simulink model "Motor_Models_Graduate_Version"  (R2024a)
settings: Solver=ode4  StartTime=0.0  StopTime=3  FixedStep=1/100  RelTol=1e-3  EnableMultiTasking=on
values from neighbouring files (symbols this model uses):
  Qvec = [-0.0101196491827 1.20927201569e-05 9.11792925381e-05 1.17252742353e-08 5.75013593968e-07 -0.000975617971472 2.07457043216e-13 -4.13179301718e-11 1.27812382623e-08 -8.38050058102e-06]    [PropData_16x55MR.mat]
undefined symbols (not defined in the file or in its folder): results_table, Vehicle
libraries: simulink_extras x1, slpidlib x1, aerolibanimutils x1
settings Model: xpc_rtwmakecfg_data=_xpciplib__xpcetherlib__xpcether8255xlib__xpcetherGbElib_  Creator=Omkar  LastModifiedBy=Teama
settings SolverCC: AlgebraicLoopSolver=TrustRegion  AutoInsertRateTranBlk=on
settings DataIOCC: ReturnWorkspaceOutputs=off
settings DebuggingCC: UnderSpecifiedDataTypeMsg=warning  UnconnectedInputMsg=warning  UnconnectedOutputMsg=warning  UnconnectedLineMsg=warning  UnderSpecifiedDimensionMsg=warning  ArithmeticOperatorsInVariantConditions=warning
settings ModelReferenceCC: EnableRefExpFcnMdlSchedulingChecks=on
settings SFSimCC: SimUseLocalCustomCode=off  CustomCodeUndefinedFunction=UseInterfaceOnly
settings RTWCC: RTWUseLocalCustomCode=off  GPUComputeCapability=3.5  DLArmComputeVersion=19.05

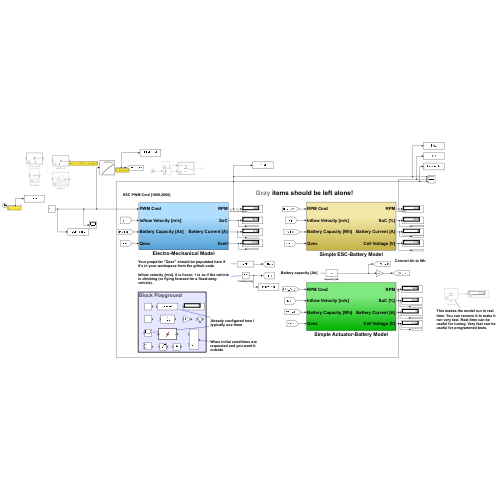
[thumbnail: Simulink's stored preview of the top-level diagram]
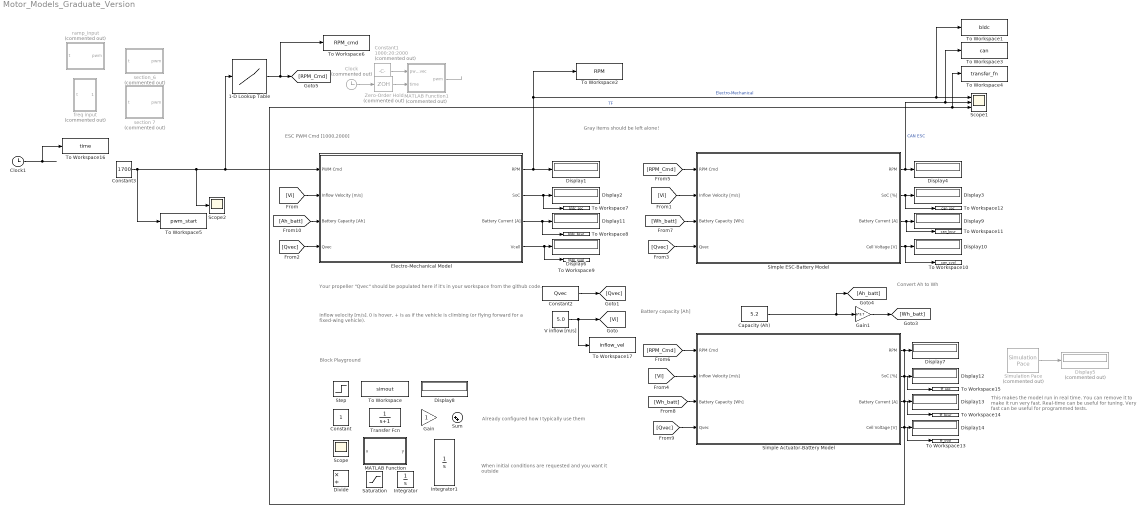
== system Motor_Models_Graduate_Version ==
  note: Block Playground
  note: Inflow velocity [m/s]. 0 is hover, + is as if the vehicle is climbing (or flying forward for a fixed-wing vehicle).
  note: Gray items should be left alone!
  note: Your propeller "Qvec" should be populated here if it's in your workspace from the github code.
  note: Battery capacity [Ah]
  note: ESC PWM Cmd [1000,2000]
  note: Already configured how I typically use them
  note: When initial conditions are requested and you want it outside
  note: This makes the model run in real time. You can remove it to make it run very fast. Real-time can be useful for tuning. Very fast can be useful for programmed tests.
  note: Convert Ah to Wh
  1-D Lookup Table : Lookup_n-D  NumberOfTableDimensions=1  BreakpointsForDimension1=results_table.pwm  Table=results_table.RPM  InternalRulePriority=Speed  RndMeth=Simplest
  Capacity (Ah) : Constant  Value=5.2
  Clock : Clock  Commented=on
  Clock1 : Clock
  Constant : Constant
  Constant1 : Constant  Commented=on  Value=1000:20:2000
  Constant2 : Constant  Value=Qvec
  Constant3 : Constant  Value=1700
  Display{1..4,6..14} (13 alike) : Display
  Display5 : Display  Commented=on
  Divide : Product  Inputs=*/
  Electro-Mechanical Model : Subsystem
  Gain : Gain
  Gain1 : Gain  Gain=6*3.7
  Integrator : Integrator
  Integrator1 : Integrator  InitialConditionSource=external
  MATLAB Function : MATLAB Function  TreatAsAtomicUnit=on
  MATLAB Function1 : MATLAB Function  Commented=on  TreatAsAtomicUnit=on
  Saturation : Saturate
  Scope : Scope
  Scope1 : Scope  NumInputPorts=3
  Scope2 : Scope
  Simple Actuator-Battery Model : Subsystem
  Simple ESC-Battery Model : Subsystem
  Simulation Pace : aerolibanimutils/Simulation Pace  Commented=on  SimulationPace=1  SleepMode=Auto  OutputPaceError=on  SampleTime=-1
  Step : Step  SampleTime=0
  Sum : Sum  Inputs=|++
  To Workspace : ToWorkspace  VariableName=simout  SampleTime=-1
      settings: Save2DSignal=2-D array (concatenate along first dimension)
  To Workspace1 : ToWorkspace  VariableName=bldc  SampleTime=-1
      settings: Save2DSignal=2-D array (concatenate along first dimension)
  To Workspace10 : ToWorkspace  VariableName=can_cvol  SampleTime=-1
      settings: Save2DSignal=2-D array (concatenate along first dimension)
  To Workspace11 : ToWorkspace  VariableName=can_bcur  SampleTime=-1
      settings: Save2DSignal=2-D array (concatenate along first dimension)
  To Workspace12 : ToWorkspace  VariableName=can_soc  SampleTime=-1
      settings: Save2DSignal=2-D array (concatenate along first dimension)
  To Workspace13 : ToWorkspace  VariableName=tf_cvol  SampleTime=-1
      settings: Save2DSignal=2-D array (concatenate along first dimension)
  To Workspace14 : ToWorkspace  VariableName=tf_bcur  SampleTime=-1
      settings: Save2DSignal=2-D array (concatenate along first dimension)
  To Workspace15 : ToWorkspace  VariableName=tf_soc  SampleTime=-1
      settings: Save2DSignal=2-D array (concatenate along first dimension)
  To Workspace16 : ToWorkspace  VariableName=time  SampleTime=-1
      settings: Save2DSignal=2-D array (concatenate along first dimension)
  To Workspace17 : ToWorkspace  VariableName=inflow_vel  SampleTime=-1
      settings: Save2DSignal=2-D array (concatenate along first dimension)
  To Workspace2 : ToWorkspace  VariableName=RPM  SampleTime=-1
      settings: Save2DSignal=2-D array (concatenate along first dimension)
  To Workspace3 : ToWorkspace  VariableName=can  SampleTime=-1
      settings: Save2DSignal=2-D array (concatenate along first dimension)
  To Workspace4 : ToWorkspace  VariableName=transfer_fn  SampleTime=-1
      settings: Save2DSignal=2-D array (concatenate along first dimension)
  To Workspace5 : ToWorkspace  VariableName=pwm_start  SampleTime=-1
      settings: Save2DSignal=2-D array (concatenate along first dimension)
  To Workspace6 : ToWorkspace  VariableName=RPM_cmd
      settings: Save2DSignal=2-D array (concatenate along first dimension)
  To Workspace7 : ToWorkspace  VariableName=bldc_soc  SampleTime=-1
      settings: Save2DSignal=2-D array (concatenate along first dimension)
  To Workspace8 : ToWorkspace  VariableName=bldc_bcur  SampleTime=-1
      settings: Save2DSignal=2-D array (concatenate along first dimension)
  To Workspace9 : ToWorkspace  VariableName=bldc_cvol  SampleTime=-1
      settings: Save2DSignal=2-D array (concatenate along first dimension)
  Transfer Fcn : TransferFcn  Denominator=[1 1]
  V inflow [m/s] : Constant  Value=5.0
  Zero-Order Hold : ZeroOrderHold  Commented=on  SampleTime=-1
  freq input : Subsystem  Commented=on
  ramp_input : MATLAB Function  Commented=on  TreatAsAtomicUnit=on
  section 7 : Subsystem  Commented=on
  section_6 : MATLAB Function  Commented=on  TreatAsAtomicUnit=on
  wires:
  Simulation Pace/1 -> Display5/1
  Electro-Mechanical Model/1(RPM) -> To Workspace1/1, Scope1/1, To Workspace2/1, Display1/1  "Electro-Mechanical"
  Electro-Mechanical Model/2(SoC) -> To Workspace7/1, Display2/1
  [RPM_Cmd] -> Simple ESC-Battery Model/1(RPM Cmd)
  Simple ESC-Battery Model/1(RPM) -> To Workspace3/1, Scope1/2, Display4/1  "CAN ESC"
  Simple ESC-Battery Model/2(SoC [%]) -> To Workspace12/1, Display3/1
  Electro-Mechanical Model/4(Vcell) -> To Workspace9/1, Display6/1
  V inflow [m/s]/1 -> To Workspace17/1, [Vi]
  [Vi] -> Electro-Mechanical Model/2(Inflow Velocity [m/s])
  [Vi] -> Simple ESC-Battery Model/2(Inflow Velocity [m/s])
  Constant2/1 -> [Qvec]
  [Qvec] -> Electro-Mechanical Model/4(Qvec)
  [Qvec] -> Simple ESC-Battery Model/4(Qvec)
  Simple ESC-Battery Model/3(Battery Current [A]) -> To Workspace11/1, Display9/1
  Simple ESC-Battery Model/4(Cell Voltage [V]) -> To Workspace10/1, Display10/1
  [RPM_Cmd] -> Simple Actuator-Battery Model/1(RPM Cmd)
  [Vi] -> Simple Actuator-Battery Model/2(Inflow Velocity [m/s])
  Capacity (Ah)/1 -> Gain1/1, [Ah_batt]
  [Wh_batt] -> Simple ESC-Battery Model/3(Battery Capacity [Wh])
  [Wh_batt] -> Simple Actuator-Battery Model/3(Battery Capacity [Wh])
  [Qvec] -> Simple Actuator-Battery Model/4(Qvec)
  Gain1/1 -> [Wh_batt]
  [Ah_batt] -> Electro-Mechanical Model/3(Battery Capacity [Ah])
  Simple Actuator-Battery Model/1(RPM) -> To Workspace4/1, Scope1/3, Display7/1  "TF"
  Electro-Mechanical Model/3(Battery Current [A]) -> To Workspace8/1, Display11/1
  Simple Actuator-Battery Model/2(SoC [%]) -> To Workspace15/1, Display12/1
  Simple Actuator-Battery Model/3(Battery Current [A]) -> To Workspace14/1, Display13/1
  Simple Actuator-Battery Model/4(Cell Voltage [V]) -> To Workspace13/1, Display14/1
  Constant1/1 -> MATLAB Function1/1(pwm_vec)
  MATLAB Function1/1(pwm) -> ?
  Clock/1 -> Zero-Order Hold/1
  Zero-Order Hold/1 -> MATLAB Function1/2(time)
  Clock1/1 -> To Workspace16/1
  Constant3/1 -> To Workspace5/1, Scope2/1, 1-D Lookup Table/1, Electro-Mechanical Model/1(PWM Cmd)
  1-D Lookup Table/1 -> To Workspace6/1, [RPM_Cmd]

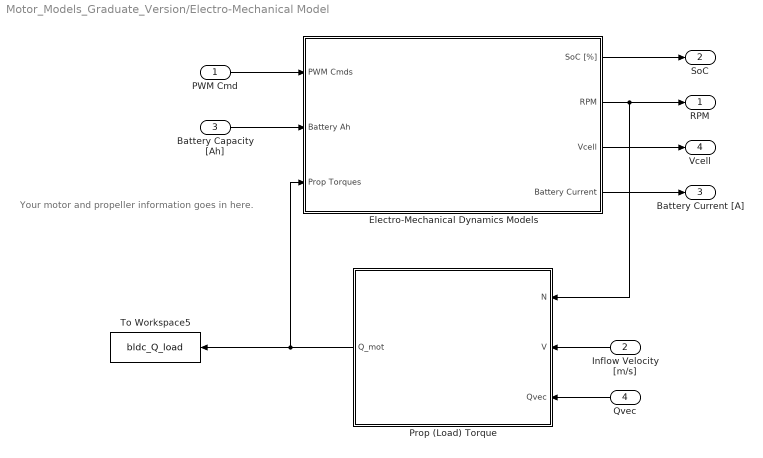
== system Motor_Models_Graduate_Version/Electro-Mechanical Model ==
  note: Your motor and propeller information goes in here.
  PWM Cmd : Inport
  Inflow Velocity [m/s] : Inport  Port=2
  Battery Capacity [Ah] : Inport  Port=3
  Qvec : Inport  Port=4
  Electro-Mechanical Dynamics Models : Subsystem
  Prop (Load) Torque : MATLAB Function  TreatAsAtomicUnit=on
  To Workspace5 : ToWorkspace  VariableName=bldc_Q_load  SampleTime=-1
      settings: Save2DSignal=2-D array (concatenate along first dimension)
  RPM : Outport
  SoC : Outport  Port=2
  Battery Current [A] : Outport  Port=3
  Vcell : Outport  Port=4
  wires:
  Prop (Load) Torque/1(Q_mot) -> To Workspace5/1, Electro-Mechanical Dynamics Models/3(Prop Torques)
  Qvec/1 -> Prop (Load) Torque/3(Qvec)
  Electro-Mechanical Dynamics Models/2(RPM) -> Prop (Load) Torque/1(N), RPM/1
  Electro-Mechanical Dynamics Models/1(SoC [%]) -> SoC/1
  PWM Cmd/1 -> Electro-Mechanical Dynamics Models/1(PWM Cmds)
  Inflow Velocity [m/s]/1 -> Prop (Load) Torque/2(V)
  Electro-Mechanical Dynamics Models/3(Vcell) -> Vcell/1
  Battery Capacity [Ah]/1 -> Electro-Mechanical Dynamics Models/2(Battery Ah)
  Electro-Mechanical Dynamics Models/4(Battery Current) -> Battery Current [A]/1

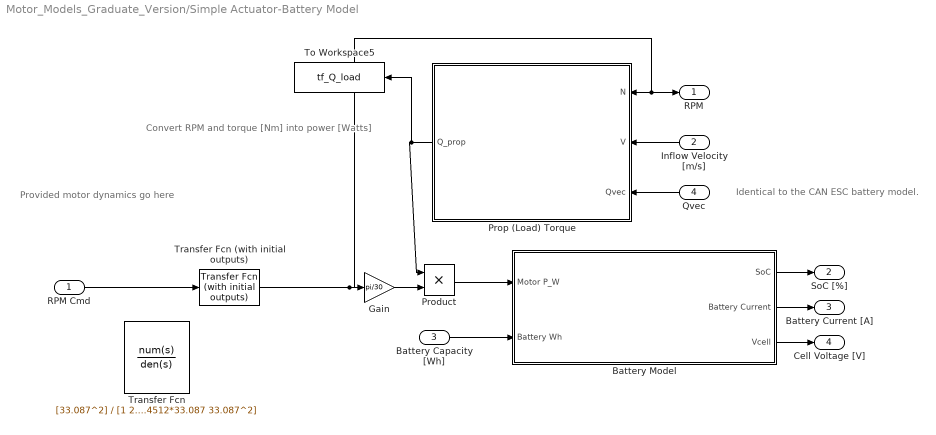
== system Motor_Models_Graduate_Version/Simple Actuator-Battery Model ==
  note: Identical to the CAN ESC battery model.
  note: Provided motor dynamics go here
  note: Convert RPM and torque [Nm] into power [Watts]
  RPM Cmd : Inport
  Inflow Velocity [m/s] : Inport  Port=2
  Battery Capacity [Wh] : Inport  Port=3
  Qvec : Inport  Port=4
  Battery Model : Subsystem
  Gain : Gain  Gain=pi/30
  Product : Product
  Prop (Load) Torque : MATLAB Function  TreatAsAtomicUnit=on
  To Workspace5 : ToWorkspace  VariableName=tf_Q_load  SampleTime=-1
      settings: Save2DSignal=2-D array (concatenate along first dimension)
  Transfer Fcn : TransferFcn  Numerator=[33.087^2]  Denominator=[1 2*1.4512*33.087 33.087^2]
  Transfer Fcn (with initial outputs) : simulink_extras/Additional Linear/Transfer Fcn (with initial outputs)  N=[33.087^2]  D=[1 2*1.4512*33.087 33.087^2]  Y0=0  U0=0
  RPM : Outport
  SoC [%] : Outport  Port=2
  Battery Current [A] : Outport  Port=3
  Cell Voltage [V] : Outport  Port=4
  wires:
  Battery Model/3(Vcell) -> Cell Voltage [V]/1
  Prop (Load) Torque/1(Q_prop) -> To Workspace5/1, Product/1
  Battery Model/2(Battery Current) -> Battery Current [A]/1
  Qvec/1 -> Prop (Load) Torque/3(Qvec)
  Inflow Velocity [m/s]/1 -> Prop (Load) Torque/2(V)
  Battery Model/1(SoC) -> SoC [%]/1
  Transfer Fcn (with initial outputs)/1 -> RPM/1, Prop (Load) Torque/1(N), Gain/1
  Product/1 -> Battery Model/1(Motor P_W)
  Battery Capacity [Wh]/1 -> Battery Model/2(Battery Wh)
  RPM Cmd/1 -> Transfer Fcn (with initial outputs)/1
  Gain/1 -> Product/2

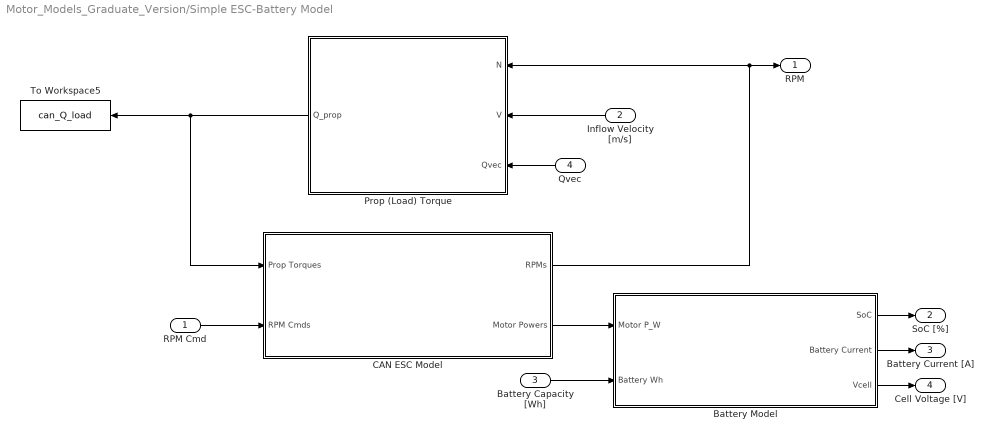
== system Motor_Models_Graduate_Version/Simple ESC-Battery Model ==
  RPM Cmd : Inport
  Inflow Velocity [m/s] : Inport  Port=2
  Battery Capacity [Wh] : Inport  Port=3
  Qvec : Inport  Port=4
  Battery Model : Subsystem
  CAN ESC Model : Subsystem
  Prop (Load) Torque : MATLAB Function  TreatAsAtomicUnit=on
  To Workspace5 : ToWorkspace  VariableName=can_Q_load  SampleTime=-1
      settings: Save2DSignal=2-D array (concatenate along first dimension)
  RPM : Outport
  SoC [%] : Outport  Port=2
  Battery Current [A] : Outport  Port=3
  Cell Voltage [V] : Outport  Port=4
  wires:
  Battery Capacity [Wh]/1 -> Battery Model/2(Battery Wh)
  CAN ESC Model/2(Motor Powers) -> Battery Model/1(Motor P_W)
  CAN ESC Model/1(RPMs) -> RPM/1, Prop (Load) Torque/1(N)
  Battery Model/1(SoC) -> SoC [%]/1
  Inflow Velocity [m/s]/1 -> Prop (Load) Torque/2(V)
  Qvec/1 -> Prop (Load) Torque/3(Qvec)
  Battery Model/2(Battery Current) -> Battery Current [A]/1
  Prop (Load) Torque/1(Q_prop) -> To Workspace5/1, CAN ESC Model/1(Prop Torques)
  RPM Cmd/1 -> CAN ESC Model/2(RPM Cmds)
  Battery Model/3(Vcell) -> Cell Voltage [V]/1

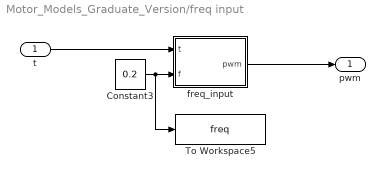
== system Motor_Models_Graduate_Version/freq input ==
  t : Inport
  Constant3 : Constant  Value=0.2
  To Workspace5 : ToWorkspace  VariableName=freq  SampleTime=-1
      settings: Save2DSignal=2-D array (concatenate along first dimension)
  freq_input : MATLAB Function  TreatAsAtomicUnit=on
  pwm : Outport
  wires:
  Constant3/1 -> To Workspace5/1, freq_input/2(f)
  freq_input/1(pwm) -> pwm/1
  t/1 -> freq_input/1(t)

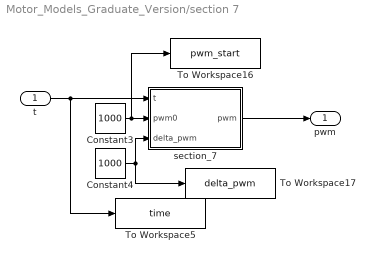
== system Motor_Models_Graduate_Version/section 7 ==
  t : Inport
  Constant3 : Constant  Value=1000
  Constant4 : Constant  Value=1000
  To Workspace16 : ToWorkspace  VariableName=pwm_start  SampleTime=-1
      settings: Save2DSignal=2-D array (concatenate along first dimension)
  To Workspace17 : ToWorkspace  VariableName=delta_pwm  SampleTime=-1
      settings: Save2DSignal=2-D array (concatenate along first dimension)
  To Workspace5 : ToWorkspace  VariableName=time  SampleTime=-1
      settings: Save2DSignal=2-D array (concatenate along first dimension)
  section_7 : MATLAB Function  TreatAsAtomicUnit=on
  pwm : Outport
  wires:
  t/1 -> section_7/1(t), To Workspace5/1
  section_7/1(pwm) -> pwm/1
  Constant4/1 -> section_7/3(delta_pwm), To Workspace17/1
  Constant3/1 -> To Workspace16/1, section_7/2(pwm0)

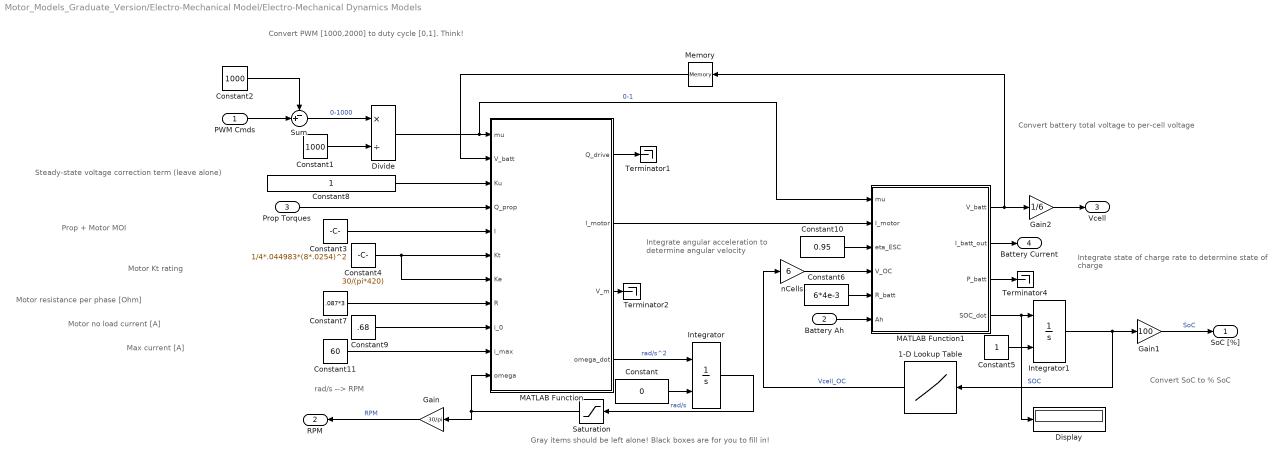
== system Motor_Models_Graduate_Version/Electro-Mechanical Model/Electro-Mechanical Dynamics Models ==
  note: Gray items should be left alone!
      | Black boxes are for you to fill in!
  note: Convert battery total voltage to per-cell voltage
  note: Integrate state of charge rate to determine state of charge
  note: Steady-state voltage correction term (leave alone)
  note: Convert PWM [1000,2000] to duty cycle [0,1]. Think!
  note: Prop + Motor MOI
  note: Motor Kt rating
  note: Motor resistance per phase [Ohm]
  note: Motor no load current [A]
  note: Max current [A]
  note: Integrate angular acceleration to determine angular velocity
  note: Convert SoC to % SoC
  note: rad/s --> RPM
  PWM Cmds : Inport
  Battery Ah : Inport  Port=2
  Prop Torques : Inport  Port=3
  1-D Lookup Table : Lookup_n-D  NumberOfTableDimensions=1  BreakpointsForDimension1="[0    0.05  0.10  0.20  0.30  0.40  0.50  0.60  0.70  0.80  0.90  1.00]"  Table="[3.20 3.45  3.55  3.65  3.70  3.74  3.77  3.80  3.84  3.90  4.00  4.20]"  InternalRulePriority=Speed  RndMeth=Simplest
  Constant : Constant  Value=0
  Constant1 : Constant  Value=1000
  Constant10 : Constant  Value=0.95
  Constant11 : Constant  Value=60
  Constant2 : Constant  Value=1000
  Constant3 : Constant  Value=1/4*.044983*(8*.0254)^2
  Constant4 : Constant  Value=30/(pi*420)
  Constant5 : Constant
  Constant6 : Constant  Value=6*4e-3
  Constant7 : Constant  Value=.087*3
  Constant8 : Constant
  Constant9 : Constant  Value=.68
  Display : Display
  Divide : Product  Inputs=*/
  Gain : Gain  Gain=30/pi
  Gain1 : Gain  Gain=100
  Gain2 : Gain  Gain=1/6
  Integrator : Integrator  InitialConditionSource=external
  Integrator1 : Integrator  InitialConditionSource=external
  MATLAB Function : MATLAB Function  TreatAsAtomicUnit=on
  MATLAB Function1 : MATLAB Function  TreatAsAtomicUnit=on
  Memory : Memory  InitialCondition=25.2
  Saturation : Saturate  UpperLimit=inf  LowerLimit=0
  Sum : Sum  Inputs=-+|
  Terminator1 : Terminator
  Terminator2 : Terminator
  Terminator4 : Terminator
  nCells : Gain  Gain=6
  SoC [%] : Outport
  RPM : Outport  Port=2
  Vcell : Outport  Port=3
  Battery Current : Outport  Port=4
  wires:
  Battery Ah/1 -> MATLAB Function1/6(Ah)
  MATLAB Function1/4(SOC_dot) -> Display/1, Integrator1/1
  Divide/1 -> MATLAB Function1/1(mu), MATLAB Function/1(mu)  "0-1"
  Integrator/1 -> Saturation/1  "rad/s"
  Constant10/1 -> MATLAB Function1/3(eta_ESC)
  Integrator1/1 -> Gain1/1, 1-D Lookup Table/1  "SOC"
  Constant3/1 -> MATLAB Function/5(I)
  Constant/1 -> Integrator/2
  Constant6/1 -> MATLAB Function1/5(R_batt)
  MATLAB Function/4(omega_dot) -> Integrator/1  "rad/s^2"
  nCells/1 -> MATLAB Function1/4(V_OC)
  MATLAB Function/3(V_m) -> Terminator2/1
  1-D Lookup Table/1 -> nCells/1  "Vcell_OC"
  Constant5/1 -> Integrator1/2
  Prop Torques/1 -> MATLAB Function/4(Q_prop)
  Constant4/1 -> MATLAB Function/7(Ke), MATLAB Function/6(Kt)
  Constant7/1 -> MATLAB Function/8(R)
  Constant9/1 -> MATLAB Function/9(i_0)
  Constant11/1 -> MATLAB Function/10(i_max)
  Gain/1 -> RPM/1  "RPM"
  Constant8/1 -> MATLAB Function/3(Ku)
  Sum/1 -> Divide/1  "0-1000"
  Constant1/1 -> Divide/2
  Constant2/1 -> Sum/1
  PWM Cmds/1 -> Sum/2
  Gain1/1 -> SoC [%]/1  "SoC"
  MATLAB Function/2(I_motor) -> MATLAB Function1/2(I_motor)
  MATLAB Function1/3(P_batt) -> Terminator4/1
  MATLAB Function1/1(V_batt) -> Gain2/1, Memory/1
  MATLAB Function/1(Q_drive) -> Terminator1/1
  Gain2/1 -> Vcell/1
  MATLAB Function1/2(I_batt_out) -> Battery Current/1
  Memory/1 -> MATLAB Function/2(V_batt)
  Saturation/1 -> Gain/1, MATLAB Function/11(omega)

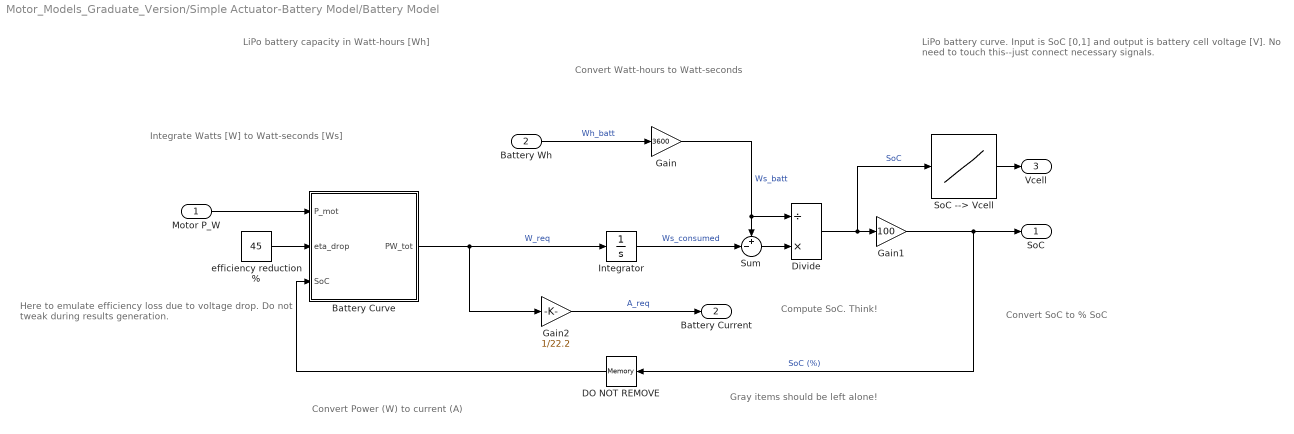
== system Motor_Models_Graduate_Version/Simple Actuator-Battery Model/Battery Model ==
  note: Gray items should be left alone!
  note: Integrate Watts [W] to Watt-seconds [Ws]
  note: Here to emulate efficiency loss due to voltage drop. Do not tweak during results generation.
  note: Convert Power (W) to current (A)
  note: Convert SoC to % SoC
  note: Convert Watt-hours to Watt-seconds
  note: LiPo battery capacity in Watt-hours [Wh]
  note: LiPo battery curve. Input is SoC [0,1] and output is battery cell voltage [V]. No need to touch this--just connect necessary signals.
  note: Compute SoC. Think!
  Motor P_W : Inport
  Battery Wh : Inport  Port=2
  Battery Curve : MATLAB Function  TreatAsAtomicUnit=on
  DO NOT REMOVE : Memory  InitialCondition=100
  Divide : Product  Inputs=/*
  Gain : Gain  Gain=3600
  Gain1 : Gain  Gain=100
  Gain2 : Gain  Gain=1/22.2
  Integrator : Integrator
  SoC --> Vcell : Lookup_n-D  NumberOfTableDimensions=1  BreakpointsForDimension1="[0    0.05  0.10  0.20  0.30  0.40  0.50  0.60  0.70  0.80  0.90  1.00]"  Table="[3.20 3.45  3.55  3.65  3.70  3.74  3.77  3.80  3.84  3.90  4.00  4.20]"  InternalRulePriority=Speed  RndMeth=Simplest
  Sum : Sum  Inputs=+-|
  efficiency reduction % : Constant  Value=45
  SoC : Outport
  Battery Current : Outport  Port=2
  Vcell : Outport  Port=3
  wires:
  SoC --> Vcell/1 -> Vcell/1
  Gain2/1 -> Battery Current/1  "A_req"
  efficiency reduction %/1 -> Battery Curve/2(eta_drop)
  DO NOT REMOVE/1 -> Battery Curve/3(SoC)
  Battery Curve/1(PW_tot) -> Gain2/1, Integrator/1  "W_req"
  Gain/1 -> Divide/1, Sum/1  "Ws_batt"
  Gain1/1 -> SoC/1, DO NOT REMOVE/1  "SoC (%)"
  Divide/1 -> SoC --> Vcell/1, Gain1/1  "SoC"
  Integrator/1 -> Sum/2  "Ws_consumed"
  Sum/1 -> Divide/2
  Motor P_W/1 -> Battery Curve/1(P_mot)
  Battery Wh/1 -> Gain/1  "Wh_batt"

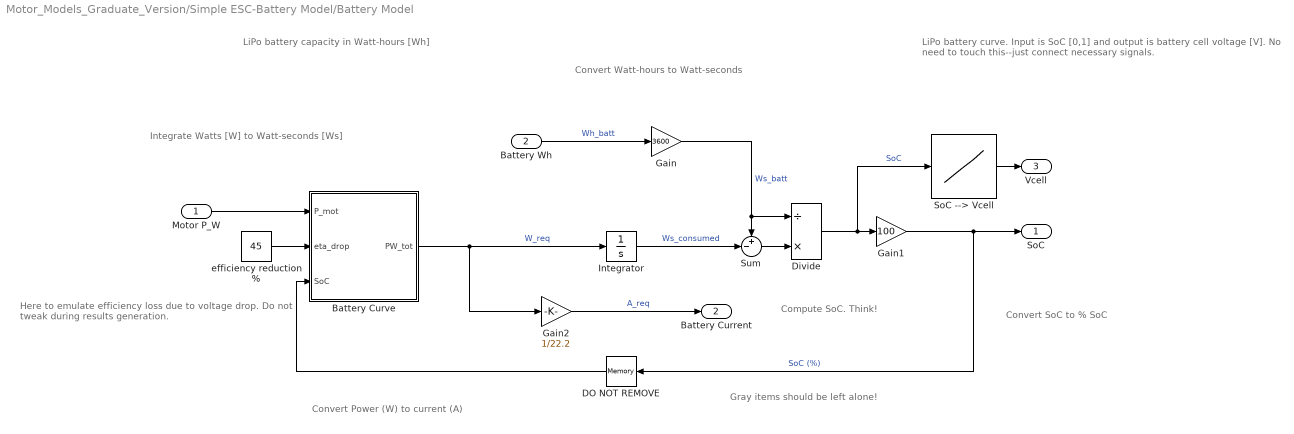
== system Motor_Models_Graduate_Version/Simple ESC-Battery Model/Battery Model ==
  note: Gray items should be left alone!
  note: Integrate Watts [W] to Watt-seconds [Ws]
  note: Here to emulate efficiency loss due to voltage drop. Do not tweak during results generation.
  note: Convert Power (W) to current (A)
  note: Convert SoC to % SoC
  note: Convert Watt-hours to Watt-seconds
  note: LiPo battery capacity in Watt-hours [Wh]
  note: LiPo battery curve. Input is SoC [0,1] and output is battery cell voltage [V]. No need to touch this--just connect necessary signals.
  note: Compute SoC. Think!
  Motor P_W : Inport
  Battery Wh : Inport  Port=2
  Battery Curve : MATLAB Function  TreatAsAtomicUnit=on
  DO NOT REMOVE : Memory  InitialCondition=100
  Divide : Product  Inputs=/*
  Gain : Gain  Gain=3600
  Gain1 : Gain  Gain=100
  Gain2 : Gain  Gain=1/22.2
  Integrator : Integrator
  SoC --> Vcell : Lookup_n-D  NumberOfTableDimensions=1  BreakpointsForDimension1="[0    0.05  0.10  0.20  0.30  0.40  0.50  0.60  0.70  0.80  0.90  1.00]"  Table="[3.20 3.45  3.55  3.65  3.70  3.74  3.77  3.80  3.84  3.90  4.00  4.20]"  InternalRulePriority=Speed  RndMeth=Simplest
  Sum : Sum  Inputs=+-|
  efficiency reduction % : Constant  Value=45
  SoC : Outport
  Battery Current : Outport  Port=2
  Vcell : Outport  Port=3
  wires:
  SoC --> Vcell/1 -> Vcell/1
  Gain2/1 -> Battery Current/1  "A_req"
  efficiency reduction %/1 -> Battery Curve/2(eta_drop)
  DO NOT REMOVE/1 -> Battery Curve/3(SoC)
  Battery Curve/1(PW_tot) -> Gain2/1, Integrator/1  "W_req"
  Gain/1 -> Divide/1, Sum/1  "Ws_batt"
  Gain1/1 -> SoC/1, DO NOT REMOVE/1  "SoC (%)"
  Divide/1 -> SoC --> Vcell/1, Gain1/1  "SoC"
  Integrator/1 -> Sum/2  "Ws_consumed"
  Sum/1 -> Divide/2
  Motor P_W/1 -> Battery Curve/1(P_mot)
  Battery Wh/1 -> Gain/1  "Wh_batt"

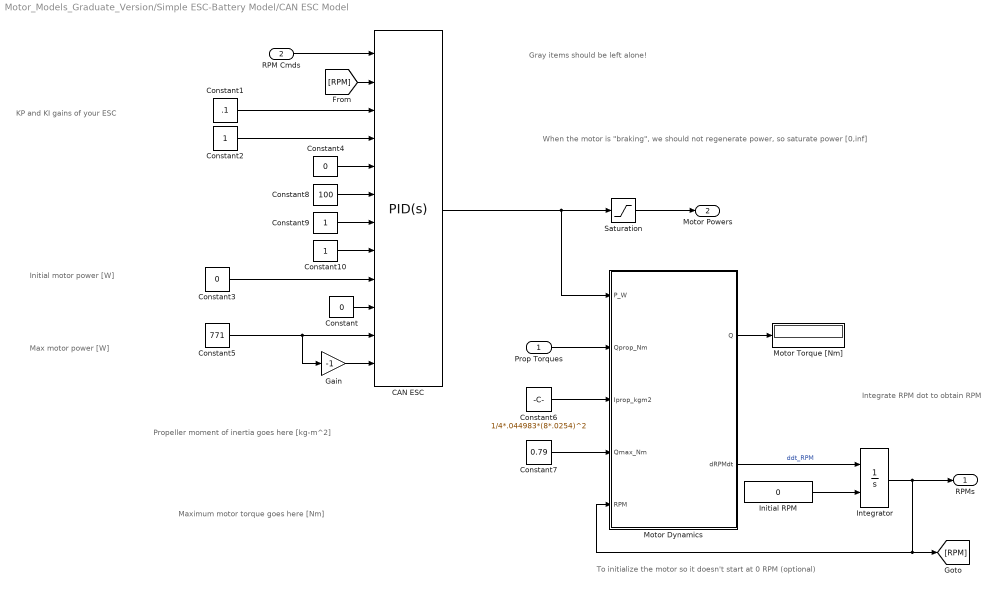
== system Motor_Models_Graduate_Version/Simple ESC-Battery Model/CAN ESC Model ==
  note: Propeller moment of inertia goes here [kg-m^2]
  note: Maximum motor torque goes here [Nm]
  note: To initialize the motor so it doesn't start at 0 RPM (optional)
  note: Max motor power [W]
  note: Initial motor power [W]
  note: KP and KI gains
      | of your ESC
  note: Gray items should be left alone!
  note: When the motor is "braking", we should not regenerate power, so saturate power [0,inf]
  note: Integrate RPM dot to obtain RPM
  Prop Torques : Inport
  RPM Cmds : Inport  Port=2
  CAN ESC : slpidlib/PID Controller (2DOF)  Controller=PID  Form=Parallel  TimeDomain=Continuous-time  UseExternalTs=off  SampleTime=-1  IntegratorMethod=Forward Euler  FilterMethod=Forward Euler  ControllerParametersSource=external  P=Vehicle.Controls.ESC.KP_LP  I=Vehicle.Controls.ESC.KI_LP  UseKiTs=off  D=0  UseExternalDerivativeSource=off  N=100  UseFilter=on  b=1  c=0  TunerSelectOption=Transfer Function Based (PID Tuner App)  InitialConditionSource=external  InitialConditionForIntegrator=0  InitialConditionForFilter=0  DifferentiatorICPrevScaledInput=0  ExternalReset=none  TrackingMode=off  Kt=1  LimitOutput=on  SatLimitsSource=external  UpperSaturationLimit=16e3  LowerSaturationLimit=-16e3  LinearizeAsGain=on  AntiWindupMode=clamping  Kb=1  LimitIntegrator=off  UpperIntegratorSaturationLimit=inf  LowerIntegratorSaturationLimit=-inf  POutMin=[]  POutMax=[]  IOutMin=[]  IOutMax=[]  DOutMin=[]  DOutMax=[]  NOutMin=[]  NOutMax=[]  bOutMin=[]  bOutMax=[]  cOutMin=[]  cOutMax=[]  SumOutMin=[]  SumOutMax=[]  SaturationOutMin=[]  SaturationOutMax=[]  PParamMin=[]  PParamMax=[]  IParamMin=[]  IParamMax=[]  DParamMin=[]  DParamMax=[]  NParamMin=[]  NParamMax=[]  bParamMin=[]  bParamMax=[]  cParamMin=[]  cParamMax=[]  KbParamMin=[]  KbParamMax=[]  KtParamMin=[]  KtParamMax=[]  KbOutMin=[]  KbOutMax=[]  KtOutMin=[]  KtOutMax=[]  IntegratorOutMin=[]  IntegratorOutMax=[]  FilterOutMin=[]  FilterOutMax=[]  SumI1OutMin=[]  SumI1OutMax=[]  SumI2OutMin=[]  SumI2OutMax=[]  SumI3OutMin=[]  SumI3OutMax=[]  SumI4OutMin=[]  SumI4OutMax=[]  SumDOutMin=[]  SumDOutMax=[]  Sum1OutMin=[]  Sum1OutMax=[]  Sum2OutMin=[]  Sum2OutMax=[]  Sum3OutMin=[]  Sum3OutMax=[]  DifferentiatorOutMin=[]  DifferentiatorOutMax=[]  FilterDiffOutCoefMin=[]  FilterDiffOutCoefMax=[]  ReciprocalOutMin=[]  ReciprocalOutMax=[]  SumDenOutMin=[]  SumDenOutMax=[]  SumNumOutMin=[]  SumNumOutMax=[]  DivideOutMin=[]  DivideOutMax=[]  UdiffTsProdOutMin=[]  UdiffTsProdOutMax=[]  NTsProdOutMin=[]  NTsProdOutMax=[]  UintegralTsProdOutMin=[]  UintegralTsProdOutMax=[]  UngainTsProdOutMin=[]  UngainTsProdOutMax=[]  ClampingZeroOutDataTypeStr=Inherit: Inherit via back propagation  ClampingZeroOutMin=[]  ClampingZeroOutMax=[]  FilterDenConstantOutDataTypeStr=Inherit: Inherit via back propagation  FilterDenConstantOutMin=[]  FilterDenConstantOutMax=[]  PCopyOutDataTypeStr=Inherit: Inherit via back propagation  PCopyOutMin=[]  PCopyOutMax=[]  NCopyOutDataTypeStr=Inherit: Inherit via back propagation  NCopyOutMin=[]  NCopyOutMax=[]  IntegratorContinuousStateAttributes=''  IntegratorStateMustResolveToSignalObject=off  IntegratorRTWStateStorageClass=Auto  FilterContinuousStateAttributes=''  FilterStateMustResolveToSignalObject=off  FilterRTWStateStorageClass=Auto  ParallelPVariant=ExternalParameters  IdealPVariant=Disabled  IVariant=ExternalParameters  DVariant=ExternalParameters  bVariant=ExternalParameters  cVariant=ExternalParameters  IntegratorVariant=Continuous  SatVariant=External  AWVariant=ContClampingParallel  PCopyVariant=Disabled  TRVariant=Disabled  FdbkBlocksVariant=Forward  IdealPFdbkVariant=Disabled  SatFdbkVariant=Disabled  DerivativeFilterVariant=ContFilter  NVariant=ExternalParameters  NCopyVariant=Disabled  FilterICVariant=ExternalICs  IntegratorICVariant=ExternalICs  ExternalResetVariant=Disabled  TRSumVariant=Passthrough  SumFdbkVariant=Disabled  SumVariant=Sum_PID  TsampFilterVariant=InternalTs  TsampNgainVariant=Passthrough  TsampIntegralVariant=Disabled_SignalSpec  ExternalSaturationOutDataTypeStr=Inherit: Same as second input  DerivativeSourceVariant=ErrorSignal
  Constant : Constant  Value=0
  Constant1 : Constant  Value=.1
  Constant10 : Constant
  Constant2 : Constant
  Constant3 : Constant  Value=0
  Constant4 : Constant  Value=0
  Constant5 : Constant  Value=771
  Constant6 : Constant  Value=1/4*.044983*(8*.0254)^2
  Constant7 : Constant  Value=0.79
  Constant8 : Constant  Value=100
  Constant9 : Constant
  Gain : Gain  Gain=-1
  Initial RPM : Constant  Value=0
  Integrator : Integrator  InitialConditionSource=external
  Motor Dynamics : MATLAB Function  TreatAsAtomicUnit=on
  Motor Torque [Nm] : Display
  Saturation : Saturate  UpperLimit=inf  LowerLimit=0
  RPMs : Outport
  Motor Powers : Outport  Port=2
  wires:
  Constant/1 -> CAN ESC/10
  Constant3/1 -> CAN ESC/9
  Integrator/1 -> Motor Dynamics/5(RPM), [RPM], RPMs/1
  RPM Cmds/1 -> CAN ESC/1
  Constant7/1 -> Motor Dynamics/4(Qmax_Nm)
  Prop Torques/1 -> Motor Dynamics/2(Qprop_Nm)
  Initial RPM/1 -> Integrator/2
  Constant6/1 -> Motor Dynamics/3(Iprop_kgm2)
  CAN ESC/1 -> Motor Dynamics/1(P_W), Saturation/1
  Motor Dynamics/2(dRPMdt) -> Integrator/1  "ddt_RPM"
  Motor Dynamics/1(Q) -> Motor Torque [Nm]/1
  Gain/1 -> CAN ESC/12
  Constant5/1 -> Gain/1, CAN ESC/11
  Constant4/1 -> CAN ESC/5
  Constant2/1 -> CAN ESC/4
  Constant1/1 -> CAN ESC/3
  [RPM] -> CAN ESC/2
  Saturation/1 -> Motor Powers/1
  Constant8/1 -> CAN ESC/6
  Constant9/1 -> CAN ESC/7
  Constant10/1 -> CAN ESC/8

== matlab function Motor_Models_Graduate_Version/section 7/section_7 ==
  data: t input; pwm output; pwm0 input; delta_pwm input
function pwm = fcn(t, pwm0, delta_pwm)
    switch true
        case t >= 0 && t < 2
            pwm = pwm0;
        case t >= 2 && t < 5
            pwm = pwm0 + delta_pwm;
        case t >= 5 && t < 8
            pwm = pwm0;
        otherwise
            pwm = pwm0;
    end
end

== matlab function Motor_Models_Graduate_Version/freq input/freq_input ==
  data: t input; pwm output; f input
function pwm = fcn(t, f)
    switch true
        case t >= 0 && t < 2
            pwm = 1650;
        otherwise
            pwm = 1650 + 50 * sin(2 * pi * f * t);
    end
end

== matlab function Motor_Models_Graduate_Version/ramp_input ==
  data: t input; pwm output
function pwm = fcn(t)
    switch true
        case t >= 0 && t < 2
            pwm = 1300;

        case t >= 2 && t < 7.0
            pwm = 1300 + ((1900 - 1300) / (7 - 2)) * (t - 2);
        case t >= 7.0 && t < 9.0
            pwm = 1900;
        case t >= 9.0 && t < 14.0
            pwm = 1900 + ((1300 - 1900) / (14 - 9)) * (t - 9);
        case t >= 14.0 && t < 16.0
            pwm = 1300;
        otherwise
            pwm = 1300
    end
end

== matlab function Motor_Models_Graduate_Version/Electro-Mechanical Model/Electro-Mechanical Dynamics Models/MATLAB Function ==
  data: mu input; Q_drive output; V_batt input; Ku input; Q_prop input; I input; Kt input; Ke input; R input; i_0 input; i_max input; omega input; I_motor output; V_m output; omega_dot output
function [Q_drive,I_motor,V_m,omega_dot] = MotorDynamics(mu,V_batt,Ku,Q_prop,I,Kt,Ke,R,i_0,i_max,omega)

    % initialize outputs
    Q_drive = 0;
    I_motor = 0;
    V_m = 0;
    omega_dot = 0;
    
    % your code goes below:
    mu_e = min(max(mu, 0), 1);

    V_m = Ku .* mu_e .* V_batt;
    
    I_motor = (V_m - Ke .* omega) ./ R;
    
    I_motor = min(max(I_motor, 0), i_max);
    
    Q_drive = Kt .* (I_motor - i_0);
    omega_dot =  (Q_drive - Q_prop) ./ I;
end

== matlab function Motor_Models_Graduate_Version/Electro-Mechanical Model/Electro-Mechanical Dynamics Models/MATLAB Function1 ==
  data: mu input; I_motor input; eta_ESC input; V_batt output; I_batt_out output; P_batt output; V_OC input; R_batt input; SOC_dot output; Ah input
function [V_batt,I_batt_out,P_batt,SOC_dot] = BatterySag(mu,I_motor,eta_ESC,V_OC,R_batt,Ah)

% initialize outputs
I_batt_out = 0;
V_batt = 0;
P_batt = 0;
SOC_dot = 0;

% your code goes below:

I_batt_out = (mu .* I_motor) ./ eta_ESC;
V_batt = max(V_OC - I_batt_out .* R_batt, 0);
P_batt = I_batt_out .* V_batt;
SOC_dot = -I_batt_out ./ (3600 * Ah);

end

== matlab function Motor_Models_Graduate_Version/Simple ESC-Battery Model/Prop (Load) Torque ==
  data: N input; Q_prop output; V input; Qvec input
function Q_prop = fcn(N,V,Qvec)

% execute the response surface equation
Q_prop =   Qvec(1) +...
            Qvec(2).*N +...
            Qvec(3).*V +...
            Qvec(4).*N.^2 +...
            Qvec(5).*N.*V +...
            Qvec(6).*V.^2 +...
            Qvec(7).*N.^3 +...
            Qvec(8).*N.^2.*V +...
            Qvec(9).*N.*V.^2 +...
            Qvec(10).*V.^3;

end

== matlab function Motor_Models_Graduate_Version/MATLAB Function ==
  data: u input; y output
function y = fcn(u)

y = u;

== matlab function Motor_Models_Graduate_Version/Simple ESC-Battery Model/CAN ESC Model/Motor Dynamics ==
  data: P_W input; Qprop_Nm input; Iprop_kgm2 input; Qmax_Nm input; RPM input; Q output; dRPMdt output
function [Q,dRPMdt] = MotorDynamics(P_W,Qprop_Nm,Iprop_kgm2,Qmax_Nm,RPM)

% initialize outputs
Q = 0;
dRPMdt = 0;

% your code goes below:

omega_safe = max(2 * pi * RPM / 60, 1);
Q_raw = P_W / omega_safe;
Q = max(-Qmax_Nm, min(Q_raw, Qmax_Nm));
dOmega_dt = (Q - Qprop_Nm) / Iprop_kgm2;
dRPMdt = dOmega_dt * 60 / (2 * pi);

end

== matlab function Motor_Models_Graduate_Version/Electro-Mechanical Model/Prop (Load) Torque ==
  data: N input; Q_mot output; V input; Qvec input
function Q_mot = fcn(N,V,Qvec)

% paste the vector of coefficients here
% Qvec = [-0.01012 1.2093e-05 9.1179e-05 1.1725e-08 5.7501e-07 -0.00097562 2.0746e-13 -4.1318e-11 1.2781e-08 -8.3805e-06];

% execute the response surface equation
Q_rse =   Qvec(1) +...
            Qvec(2).*N +...
            Qvec(3).*V +...
            Qvec(4).*N.^2 +...
            Qvec(5).*N.*V +...
            Qvec(6).*V.^2 +...
            Qvec(7).*N.^3 +...
            Qvec(8).*N.^2.*V +...
            Qvec(9).*N.*V.^2 +...
            Qvec(10).*V.^3;

% correct for air density
sigma = 1;
Q_mot = Q_rse*sqrt(sigma);

end

== matlab function Motor_Models_Graduate_Version/Simple ESC-Battery Model/Battery Model/Battery Curve ==
  data: P_mot input; PW_tot output; eta_drop input; SoC input
function PW_tot = fcn(P_mot,eta_drop,SoC)

% sum all incoming prop powers
PW_tot = sum(P_mot);

% with a reduction in the state of charge, the battery becomes even less efficient
SoC_factor = 1 - 0.01*(SoC - 100);
% battery efficiency is a function of total power draw and SoC
eta = 1/100*(90 - eta_drop*SoC_factor/1000*PW_tot);
% eta should never drop below a logical value
eta = max(0.3,eta);

% account for efficiency loss
PW_tot = PW_tot/eta;

end

== matlab function Motor_Models_Graduate_Version/Simple Actuator-Battery Model/Battery Model/Battery Curve ==
  data: P_mot input; PW_tot output; eta_drop input; SoC input
function PW_tot = fcn(P_mot,eta_drop,SoC)

% sum all incoming prop powers
PW_tot = sum(P_mot);

% with a reduction in the state of charge, the battery becomes even less efficient
SoC_factor = 1 - 0.01*(SoC - 100);
% battery efficiency is a function of total power draw and SoC
eta = 1/100*(90 - eta_drop*SoC_factor/1000*PW_tot);
% eta should never drop below a logical value
eta = max(0.3,eta);

% account for efficiency loss
PW_tot = PW_tot/eta;

end

== matlab function Motor_Models_Graduate_Version/MATLAB Function1 ==
  data: pwm_vec input; pwm output; time input
function pwm = fcn(pwm_vec, time)
    persistent idx;
    persistent last_time;
    
    if isempty(idx)
        idx = 1;
    end

    if isempty(last_time)
        last_time = 0;
    end

    if (time - last_time >= 2)
        idx = idx + 1;
        last_time = time;
    end
    
    if (idx < length(pwm_vec))
        pwm = pwm_vec(idx);
    else
        pwm = pwm_vec(end);
    end

end

== matlab function Motor_Models_Graduate_Version/Simple Actuator-Battery Model/Prop (Load) Torque ==
  data: N input; Q_prop output; V input; Qvec input
function Q_prop = fcn(N,V,Qvec)

% execute the response surface equation
Q_prop =   Qvec(1) +...
            Qvec(2).*N +...
            Qvec(3).*V +...
            Qvec(4).*N.^2 +...
            Qvec(5).*N.*V +...
            Qvec(6).*V.^2 +...
            Qvec(7).*N.^3 +...
            Qvec(8).*N.^2.*V +...
            Qvec(9).*N.*V.^2 +...
            Qvec(10).*V.^3;

end

== matlab function Motor_Models_Graduate_Version/section_6 ==
  data: t input; pwm output
function pwm = fcn(t)
    switch true
        case t >= 0 && t < 2
            pwm = 1480;
        case t >= 2 && t < 4
            pwm = 1530;
        case t >= 4 && t < 6
            pwm = 1480;
        otherwise
            pwm = 1480;
    end
end
